simulink model "METODA_POLI_ZEROURI_Kp_schimbat"  (R2025b)
settings: Solver=VariableStepAuto  StartTime=0.0  StopTime=20  RelTol=1e-3
settings Model: Creator=anama  LastModifiedBy=anama

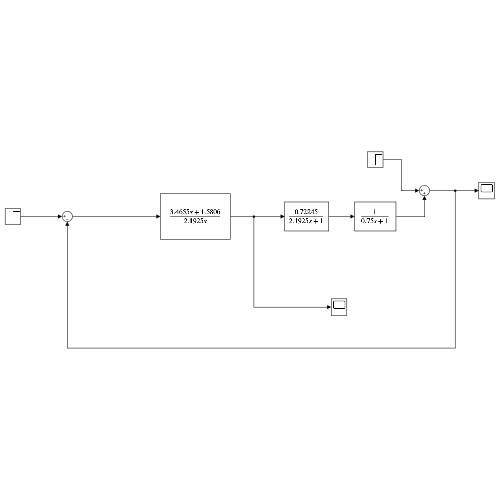
[thumbnail: Simulink's stored preview of the top-level diagram]
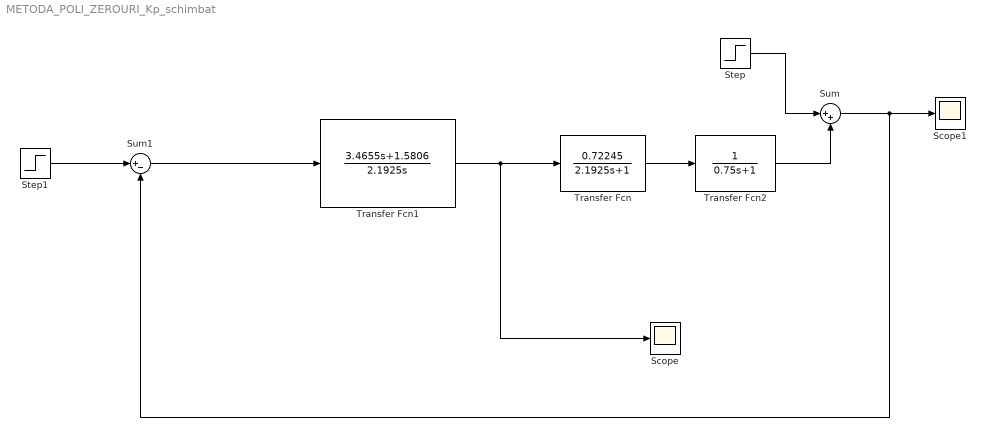
== system METODA_POLI_ZEROURI_Kp_schimbat ==
  Scope : Scope
      settings: ActiveDisplayYMinimum=233.94202825780087  ActiveDisplayYMaximum=234.03190936128757
  Scope1 : Scope
      settings: ActiveDisplayYMinimum=112.27326505373262  ActiveDisplayYMaximum=115.55833318085551
  Step : Step  Time=0  After=10  SampleTime=0
  Step1 : Step  Time=0  After=110  SampleTime=0
  Sum : Sum  Inputs=|++
  Sum1 : Sum  Inputs=|+-
  Transfer Fcn : TransferFcn  Numerator=[0.72245]  Denominator=[2.1925 1]
  Transfer Fcn1 : TransferFcn  Numerator=[3.4655 1.5806]  Denominator=[2.1925 0]
  Transfer Fcn2 : TransferFcn  Denominator=[0.75 1]
  wires:
  Transfer Fcn/1 -> Transfer Fcn2/1
  Step/1 -> Sum/1
  Transfer Fcn2/1 -> Sum/2
  Sum/1 -> Sum1/2, Scope1/1
  Transfer Fcn1/1 -> Scope/1, Transfer Fcn/1
  Sum1/1 -> Transfer Fcn1/1
  Step1/1 -> Sum1/1
